simulink model "three_phase_short_circuit"  (R2021a)
settings: Solver=VariableStepAuto  StartTime=0.0  StopTime=15  RelTol=1e-3
undefined symbols (not defined in the file): D1, Delta
libraries: spsThreePhaseSeriesRLCLoadLib x2, spsExcitationSystemLib x1, spsHydraulicTurbineandGovernorLib x1, spsSynchronousMachinepuFundamentalLib x1, spsThreePhasePISectionLineLib x1, spsThreePhaseTransformerTwoWindingsLib x1, spsThreePhaseFaultLib x1, spsThreePhaseSourceLib x1, spspowerguiLib x1
settings Model: Creator=muham  LastModifiedBy=muham

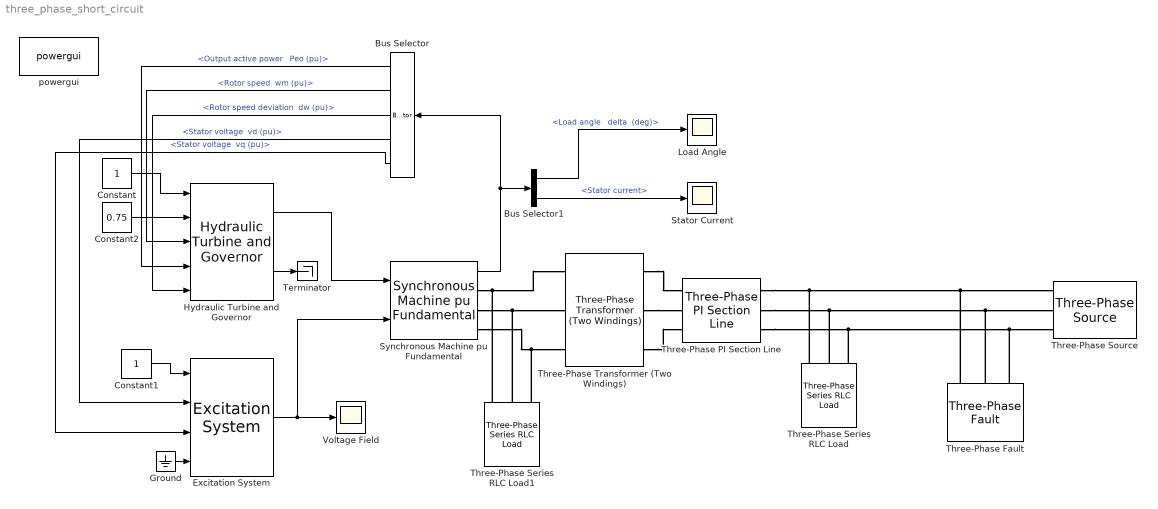
== system three_phase_short_circuit ==
  Bus Selector : BusSelector  OutputSignals="Output active power   Peo (pu),Mechanical.Rotor speed  wm (pu),Mechanical.Rotor speed deviation  dw (pu),dq0 components.Stator voltage  vd (pu),dq0 components.Stator voltage  vq (pu)"
  Bus Selector1 : BusSelector  OutputSignals="Load angle   delta  (deg),Stator current"
  Constant : Constant
  Constant1 : Constant
  Constant2 : Constant  Value=0.75
  Excitation System : spsExcitationSystemLib/Excitation System  tr=20e-3  reg=[ 300, 0.001 ]  exc=[ 1, 0 ]  tgr=[ 0, 0 ]  damp=[ 0.001, 0.1 ]  sat=[ 0, 0 ]  lim=[ -11.5, 11.5, 0 ]  v0="[1.0  1.28]"
      settings: SourceProductBaseCode=PS
  Ground : Ground
  Hydraulic Turbine and Governor : spsHydraulicTurbineandGovernorLib/Hydraulic Turbine and Governor  sm="[ 10/3  0.07 ]"  gate="[  0.01  0.97518  -0.1  0.1 ]"  reg="[  0.05  1.163  0.105  0  0.01  ]"  hyd="[  0  2.67  ]"  dref=0  po=0.7516
      settings: SourceProductBaseCode=PS
  Load Angle : Scope
  Stator Current : Scope
  Synchronous Machine pu Fundamental : spsSynchronousMachinepuFundamentalLib/Synchronous Machine pu Fundamental  PresetModel=No  MechanicalLoad=Mechanical power Pm  ShowDetailedParameters=on  RotorType=Salient-pole  Units=per unit fundamental parameters  MeasurementBus=off  NominalParameters="[ 187E6  13800   60]"  Stator="[ 2.85E-03  0.114  1.19  0.36 ]"  Field="[ 5.79E-04  0.114]"  Dampers2=[0.0652, 0.5134, 0.0287, 0.2553, 7.765e-3, 0.9167 ]  Dampers1="[ 1.17E-02  0.182  1.97E-02  0.384 ]"  Mechanical=[ 3.7 0 20]  PolePairs=20  InitialConditions="[ 0  0  0  0  0  0  0  0  1 ]"  SetSaturation=off  Saturation=[0.6404,0.7127,0.8441,0.9214,0.9956,1.082,1.19,1.316,1.457;0.7,0.7698,0.8872,0.9466,0.9969,1.046,1.1,1.151,1.201]  LoadFlowParameters=[1,0,0,0,0]  TsPowergui=0  TsBlock=-1  IterativeModel=Trapezoidal non iterative  IterativeDiscreteModel=Trapezoidal non iterative  BusType=PV  Pref=0  Qref=0  Qmin=-inf  Qmax=inf  PLF=0  QLF=0
      settings: SourceProductBaseCode=PS
  Terminator : Terminator
  Three-Phase PI Section Line : spsThreePhasePISectionLineLib/Three-Phase PI Section Line  LConnTagsString=a|b|c  RConnTagsString=A|B|C  Length=100  Frequency=60  Resistances=[ 0.01273 0.3864]  Inductances="[ 0.9337e-3  4.1264e-3]"  Capacitances=[12.74e-9 7.751e-9]
  Three-Phase Series RLC Load : spsThreePhaseSeriesRLCLoadLib/Three-Phase Series RLC Load  LConnTagsString=A|B|C  Configuration=Y (grounded)  NominalVoltage=230e3  Vabc=[1e3 1e3 1e3]  Vabcp=[1e3 1e3 1e3]  NominalFrequency=60  UnbalancedPower=off  ActivePower=10e3  InductivePower=100  CapacitivePower=100  Pabc=[10e3 9e3 11e3]  QLabc=[100 90 110]  QCabc=[100 90 110]  Pabcp=[10e3 9e3 11e3]  QLabcp=[100 90 110]  QCabcp=[100 90 110]  Measurements=None  LoadType=constant Z
  Three-Phase Series RLC Load1 : spsThreePhaseSeriesRLCLoadLib/Three-Phase Series RLC Load  LConnTagsString=A|B|C  Configuration=Y (grounded)  NominalVoltage=230e3  Vabc=[1e3 1e3 1e3]  Vabcp=[1e3 1e3 1e3]  NominalFrequency=60  UnbalancedPower=off  ActivePower=10e3  InductivePower=0  CapacitivePower=0  Pabc=[10e3 9e3 11e3]  QLabc=[100 90 110]  QCabc=[100 90 110]  Pabcp=[10e3 9e3 11e3]  QLabcp=[100 90 110]  QCabcp=[100 90 110]  Measurements=None  LoadType=constant Z
  Three-Phase Transformer (Two Windings) : spsThreePhaseTransformerTwoWindingsLib/Three-Phase Transformer (Two Windings)  Winding1Connection=Delta (D1)  Winding2Connection=Yg  CoreType=Three single-phase transformers  SetSaturation=off  Hysteresis=off  DataFile='hysteresis'  SetInitialFlux=off  Measurements=None  UNITS=pu  NominalPower=[ 250e6 , 60 ]  Winding1=[ 13.8e3 , 0.002 , 0.08 ]  Winding2=[ 230e3 , 0.002 , 0.08 ]  Rm=500  Lm=500  L0=0.5  Saturation=[ 0,0 ; 0.0024,1.2 ; 1.0,1.52 ]  InitialFluxes=[ 0.8 , -0.8 , 0.7 ]  BreakLoop=off  DiscreteSolver=Trapezoidal iterative  DataType=off  TransfoNumber=1
  Three-Phase Fault : spsThreePhaseFaultLib/Three-Phase Fault  InitialStates=0  FaultA=on  FaultB=on  FaultC=on  GroundFault=on  SwitchTimes=[.1 .2]  External=off  SwitchStatus=NaN  FaultResistance=0.001  GroundResistance=0.01  SnubberResistance=1e6  SnubberCapacitance=inf  Measurements=None
  Three-Phase Source : spsThreePhaseSourceLib/Three-Phase Source  InternalConnection=Yg  VoltagePhases=off  Voltage=230e3  PhaseAngle=0  Voltage_phases=[25e3 25e3 25e3]/sqrt(3)  PhaseAngles_phases=[0 -120 +120]  Frequency=60  NonIdealSource=on  SpecifyImpedance=off  Resistance=0.8929  Inductance=16.58e-3  ShortCircuitLevel=100e6  BaseVoltage=25e3  XRratio=7  BusType=swing  Pref=10e3  Qref=0  Prefabc=[10e3, 10e3, 10e3]  Qrefabc=[0, 0, 0]  Qmin=-inf  Qmax=inf
  Voltage Field : Scope
  powergui : spspowerguiLib/powergui  Priority=1  SimulationMode=Phasor  SampleTime=50e-6  frequency=60  Iterations=50  frequencyindice=60  Pbase=100e6  ErrMax=1e-4  UnitsV=kV  UnitsW=MW  buscounter=0  FunctionMessages=off  echomessages=off  EnableUseOfTLC=off  CurrentSourceSwitches=off  DisableSnubberDevices=off  DisableRonSwitches=off  DisableVfSwitches=off  DisplayEquations=off  AutomaticDiscreteSolvers=off  SolverType=Tustin/Backward Euler (TBE)  Interpol=off  ExternalGateDelay=off  methode=off  Ts=100  x0status=blocks  SPID=on  SwTol=0  HookPort=off  NonlinearTolerance=1e-4  nMaxIteration=100  ContinueOnMaxIteration=off  RestoreLinks=warning  ResistiveCurrentMeasurement=off  Frange=[0:2:500]  Ylog=off  Xlog=on  ShowGrid=off  save=off  variable=ZData  structure=0  ZoomFFT=off  StartTime=0.0  cycles=1  DisplayStyle=1  fundamental=60  FreqAxis=off  MaxFrequency=1000  frequencyindicesteady=1  RmsSteady=1  display=off
  wires:
  Bus Selector1/1 -> Load Angle/1  "<Load angle   delta  (deg)>"
  Bus Selector1/2 -> Stator Current/1  "<Stator current>"
  Synchronous Machine pu Fundamental/1 -> Bus Selector/1, Bus Selector1/1
  Hydraulic Turbine and Governor/1 -> Synchronous Machine pu Fundamental/1
  Constant2/1 -> Hydraulic Turbine and Governor/2
  Constant/1 -> Hydraulic Turbine and Governor/1
  Constant1/1 -> Excitation System/1
  Bus Selector/1 -> Hydraulic Turbine and Governor/4  "<Output active power   Peo (pu)>"
  Bus Selector/2 -> Hydraulic Turbine and Governor/3  "<Rotor speed  wm (pu)>"
  Bus Selector/3 -> Hydraulic Turbine and Governor/5  "<Rotor speed deviation  dw (pu)>"
  Bus Selector/4 -> Excitation System/2  "<Stator voltage  vd (pu)>"
  Bus Selector/5 -> Excitation System/3  "<Stator voltage  vq (pu)>"
  Ground/1 -> Excitation System/4
  Excitation System/1 -> Synchronous Machine pu Fundamental/2, Voltage Field/1
  Hydraulic Turbine and Governor/2 -> Terminator/1
  connections:
  Synchronous Machine pu Fundamental/RConn1 -- Three-Phase Transformer (Two Windings)/LConn1 -- Three-Phase Series RLC Load1/LConn1
  Synchronous Machine pu Fundamental/RConn2 -- Three-Phase Series RLC Load1/LConn2 -- Three-Phase Transformer (Two Windings)/LConn2
  Synchronous Machine pu Fundamental/RConn3 -- Three-Phase Series RLC Load1/LConn3 -- Three-Phase Transformer (Two Windings)/LConn3
  Three-Phase Transformer (Two Windings)/RConn1 -- Three-Phase PI Section Line/LConn1
  Three-Phase Transformer (Two Windings)/RConn2 -- Three-Phase PI Section Line/LConn2
  Three-Phase Transformer (Two Windings)/RConn3 -- Three-Phase PI Section Line/LConn3
  Three-Phase PI Section Line/RConn1 -- Three-Phase Series RLC Load/LConn1 -- Three-Phase Fault/LConn1 -- Three-Phase Source/RConn1
  Three-Phase PI Section Line/RConn2 -- Three-Phase Series RLC Load/LConn2 -- Three-Phase Source/RConn2 -- Three-Phase Fault/LConn2
  Three-Phase PI Section Line/RConn3 -- Three-Phase Series RLC Load/LConn3 -- Three-Phase Fault/LConn3 -- Three-Phase Source/RConn3
